simulink model "EINT_system_simulation"  (R2025b)
settings: Solver=FixedStepAuto  StartTime=0.0  StopTime=8  FixedStep=Ts  RelTol=1e-3
values from neighbouring files (symbols this model uses):
  Ts = 0.05    [random_init.m]
settings Model: Creator=Max  LastModifiedBy=anoua
settings SolverCC: AlgebraicLoopSolver=TrustRegion
settings DebuggingCC: UnconnectedInputMsg=warning  UnconnectedOutputMsg=warning  UnconnectedLineMsg=warning
settings ModelReferenceCC: EnableRefExpFcnMdlSchedulingChecks=on
settings RTWCC: GPUComputeCapability=3.5

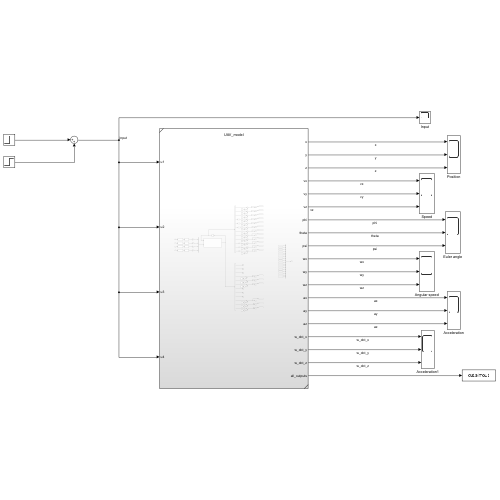
[thumbnail: Simulink's stored preview of the top-level diagram]
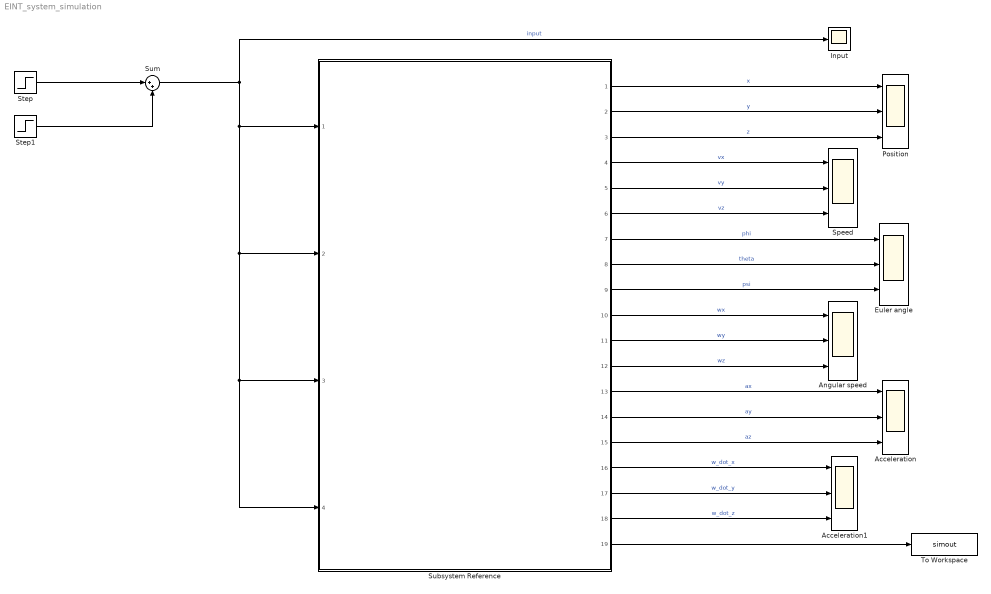
== system EINT_system_simulation ==
  Acceleration : Scope  NumInputPorts=3
      settings: ActiveDisplayYMinimum=-49.472474523205918  ActiveDisplayYMaximum=21.966976065630941
  Acceleration1 : Scope  NumInputPorts=3
      settings: ActiveDisplayYMinimum=-0.0013807612811449379  ActiveDisplayYMaximum=0.0013516531131701009  DataLoggingVariableName=ScopeData2
  Angular speed : Scope  NumInputPorts=3
      settings: ActiveDisplayYMinimum=-0.45167  ActiveDisplayYMaximum=0.49611  DataLoggingVariableName=ScopeData3
  Euler angle : Scope  NumInputPorts=3
      settings: ActiveDisplayYMinimum=-1  ActiveDisplayYMaximum=1  DataLoggingVariableName=ScopeData4
  Input : Scope
      settings: ActiveDisplayYMinimum=-1  ActiveDisplayYMaximum=1  DataLoggingVariableName=ScopeData5
  Position : Scope  NumInputPorts=3
      settings: ActiveDisplayYMinimum=-7.76558010650157  ActiveDisplayYMaximum=63.0223095668932  DataLoggingVariableName=ScopeData6
  Speed : Scope  NumInputPorts=3
      settings: ActiveDisplayYMinimum=-65.08231296474483  ActiveDisplayYMaximum=19.741944356483096
  Step : Step  Time=0  After=0.49  SampleTime=0
  Step1 : Step  Time=5  After=0  SampleTime=0
  Subsystem Reference : Subsystem  ReferencedSubsystem=UAV_model
  Sum : Sum  Inputs=|++
  To Workspace : ToWorkspace  VariableName=simout  SaveFormat=Structure With Time  SampleTime=Ts
  wires:
  Subsystem Reference/18 -> Acceleration1/3  "w_dot_z"
  Subsystem Reference/12 -> Angular speed/3  "wz"
  Subsystem Reference/17 -> Acceleration1/2  "w_dot_y"
  Subsystem Reference/9 -> Euler angle/3  "psi"
  Subsystem Reference/8 -> Euler angle/2  "theta"
  Subsystem Reference/14 -> Acceleration/2  "ay"
  Subsystem Reference/10 -> Angular speed/1  "wx"
  Subsystem Reference/2 -> Position/2  "y"
  Subsystem Reference/13 -> Acceleration/1  "ax"
  Subsystem Reference/15 -> Acceleration/3  "az"
  Subsystem Reference/16 -> Acceleration1/1  "w_dot_x"
  Subsystem Reference/7 -> Euler angle/1  "phi"
  Subsystem Reference/19 -> To Workspace/1
  Subsystem Reference/1 -> Position/1  "x"
  Subsystem Reference/6 -> Speed/3  "vz"
  Subsystem Reference/4 -> Speed/1  "vx"
  Sum/1 -> Subsystem Reference/1, Subsystem Reference/4, Subsystem Reference/3, Subsystem Reference/2, Input/1  "input"
  Subsystem Reference/3 -> Position/3  "z"
  Subsystem Reference/5 -> Speed/2  "vy"
  Subsystem Reference/11 -> Angular speed/2  "wy"
  Step/1 -> Sum/1
  Step1/1 -> Sum/2
